simulink library "ConverterLibrary"  (R2026a)
settings: Solver=VariableStepAuto
undefined symbols (not defined in the file or in its folder): DiscIntNeverNeededParam, dspblkCoreblockFVToolHelper, gcbh, gridInverter
libraries: fl_lib x240, nesl_utility x221, ee_lib x208, slpidlib x28, eeGeneralControl x12, simulink x9, eeTransforms x4, simulink_extras x1, eePowerMeasurement x1
(part 10 of 30)

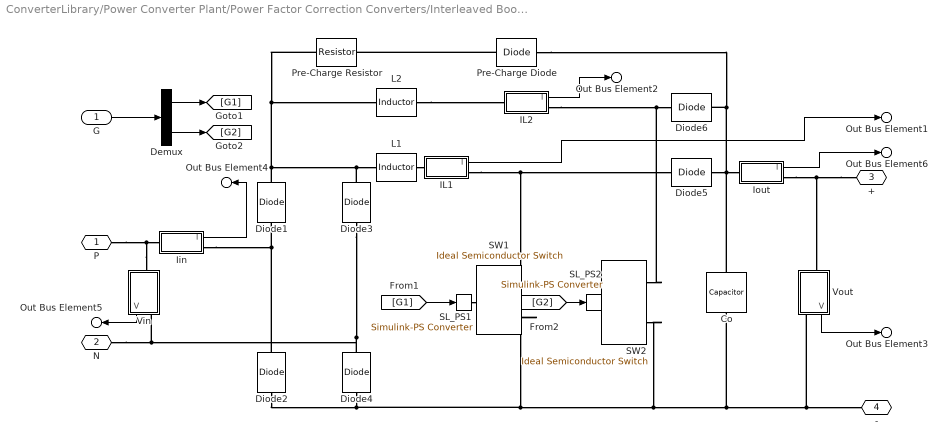
== system ConverterLibrary/Power Converter Plant/Power Factor Correction Converters/Interleaved Boost PFC Converter/InterleavedBoostPFCVariant/SimplifiedModel ==
  G : Inport
  Co : ee_lib/Passive/Capacitor  cap_option=ee.enum.passive.capacitor.capOption.const  c=CBoost_SI F  Cvec=[1e-05, 1e-06] F  Vvec=[0, 10] V  CV_table_symmetry=ee.enum.passive.capacitor.tableSymmetry.yes  f_vec=[1, 10] kHz  DFext_vec=[.8, 1.2]  enable_C_tol=ee.enum.toleranceApplication.none  averaging_period=0 s  C_tol=5  tol_distribution=ee.enum.toleranceDistribution.uniform  nSigma=4  r=Rco_SI Ohm  g=1e-05 1/Ohm  enable_operating_limits=ee.enum.enable.no  operating_limit_action=ee.enum.passive.reportOpLim.warn  max_working_voltage_range=[-25, 25] V  power_rating=1 W  maxTemperature=85 degC  thermalEnable=false  thermalMass=1 J/K  i_specify=off  i_priority=None  i=0 A  i_nominal_specify=off  i_nominal_value=1  i_nominal_unit=A  v_specify=off  v_priority=None  v=0 V  v_nominal_specify=off  v_nominal_value=1  v_nominal_unit=V  vc_specify=on  vc_priority=High  vc=Vco_SI V  vc_nominal_specify=off  vc_nominal_value=1  vc_nominal_unit=V  T_specify=off  T_priority=None  T=298.15 K  T_nominal_specify=off  T_nominal_value=1  T_nominal_unit=K
  Demux : Demux  Outputs=2
  Diode{1..4} (4 alike) : fl_lib/Electrical/Electrical Elements/Diode  Vf=VfRect_SI V  Ron=RdRect_SI Ohm  Goff=GdRect_SI 1/Ohm  i_specify=off  i_priority=None  i=0 A  i_nominal_specify=off  i_nominal_value=1  i_nominal_unit=A  v_specify=off  v_priority=None  v=0 V  v_nominal_specify=off  v_nominal_value=1  v_nominal_unit=V
  Diode5 : fl_lib/Electrical/Electrical Elements/Diode  Vf=VfDiode_SI V  Ron=RdDiode_SI Ohm  Goff=GdDiode_SI 1/Ohm  i_specify=off  i_priority=None  i=0 A  i_nominal_specify=off  i_nominal_value=1  i_nominal_unit=A  v_specify=off  v_priority=None  v=0 V  v_nominal_specify=off  v_nominal_value=1  v_nominal_unit=V
  Diode6 : fl_lib/Electrical/Electrical Elements/Diode  Vf=VfDiode_SI V  Ron=RdDiode_SI Ohm  Goff=GdDiode_SI 1/Ohm  i_specify=off  i_priority=None  i=0 A  i_nominal_specify=off  i_nominal_value=1  i_nominal_unit=A  v_specify=off  v_priority=None  v=0 V  v_nominal_specify=off  v_nominal_value=1  v_nominal_unit=V
  IL1 : Subsystem
      mask Display: disp('I')
  IL2 : Subsystem
      mask Display: disp('I')
  Iin : Subsystem
      mask Display: disp('I')
  Iout : Subsystem
      mask Display: disp('I')
  L1 : ee_lib/Passive/Inductor  l=LBoost_SI H  enable_L_tol=ee.enum.toleranceApplication.none  L_tol=20  tol_distribution=ee.enum.toleranceDistribution.uniform  nSigma=4  r=RLboost_SI Ohm  g=1e-05 1/Ohm  enable_operating_limits=ee.enum.enable.no  operating_limit_action=ee.enum.passive.reportOpLim.warn  max_working_current=1 A  power_rating=1 W  i_L_specify=off  i_L_priority=High  i_L=0 A  i_L_nominal_specify=off  i_L_nominal_value=1  i_L_nominal_unit=A
  L2 : ee_lib/Passive/Inductor  l=LBoost_SI H  enable_L_tol=ee.enum.toleranceApplication.none  L_tol=20  tol_distribution=ee.enum.toleranceDistribution.uniform  nSigma=4  r=RLboost_SI Ohm  g=1e-05 1/Ohm  enable_operating_limits=ee.enum.enable.no  operating_limit_action=ee.enum.passive.reportOpLim.warn  max_working_current=1 A  power_rating=1 W  i_L_specify=off  i_L_priority=High  i_L=0 A  i_L_nominal_specify=off  i_L_nominal_value=1  i_L_nominal_unit=A
  Pre-Charge Diode : fl_lib/Electrical/Electrical Elements/Diode  Vf=VfPreCharge_SI V  Ron=RdPreCharge_SI Ohm  Goff=GdPreCharge_SI 1/Ohm  i_specify=off  i_priority=None  i=0 A  i_nominal_specify=off  i_nominal_value=1  i_nominal_unit=A  v_specify=off  v_priority=None  v=0 V  v_nominal_specify=off  v_nominal_value=1  v_nominal_unit=V
  Pre-Charge Resistor : fl_lib/Electrical/Electrical Elements/Resistor  R=RPreCharge_SI Ohm  i_specify=off  i_priority=None  i=0 A  i_nominal_specify=off  i_nominal_value=1  i_nominal_unit=A  v_specify=off  v_priority=None  v=0 V  v_nominal_specify=off  v_nominal_value=1  v_nominal_unit=V
  SL_PS1 : nesl_utility/Simulink-PS Converter  PhysicalDomain=network_engine_domain  SubClassName=ps_input  LeftPortType=input  RightPortType=output  PseudoPeriodic=off  Frequencies=[]  NoiseDistribution=none  NoiseParameters=[]  Unit=1  AffineConversion=off  FilteringAndDerivatives=provide  SimscapeFilterOrder=1  InputFilterTimeConstant=0.001  UdotUserProvided=0
  SL_PS2 : nesl_utility/Simulink-PS Converter  PhysicalDomain=network_engine_domain  SubClassName=ps_input  LeftPortType=input  RightPortType=output  PseudoPeriodic=off  Frequencies=[]  NoiseDistribution=none  NoiseParameters=[]  Unit=1  AffineConversion=off  FilteringAndDerivatives=provide  SimscapeFilterOrder=1  InputFilterTimeConstant=0.001  UdotUserProvided=0
  SW1 : ee_lib/Semiconductors & Converters/Ideal Semiconductor Switch  port_option=ee.enum.controlport.ps  Ron=RdsOn_SI Ohm  Goff=GdsOff_SI 1/Ohm  Vth=Vth_SI V  diode_param=ee.enum.semiconductors.protectionDiode.external  diode_Vf=0.8 V  diode_Ron=0.001 Ohm  diode_Goff=1e-5 1/Ohm  diode_C=50e-9 F  diode_iRM=-235 A  diode_iF=300 A  diode_idot=-50 A/us  diode_trr_param=ee.enum.converters.diodetrr.trr_factor  diode_trr_factor=3  diode_trr=15 us  diode_Qrr=1500 s*uA
  SW2 : ee_lib/Semiconductors & Converters/Ideal Semiconductor Switch  port_option=ee.enum.controlport.ps  Ron=RdsOn_SI Ohm  Goff=GdsOff_SI 1/Ohm  Vth=Vth_SI V  diode_param=ee.enum.semiconductors.protectionDiode.external  diode_Vf=0.8 V  diode_Ron=0.001 Ohm  diode_Goff=1e-5 1/Ohm  diode_C=50e-9 F  diode_iRM=-235 A  diode_iF=300 A  diode_idot=-50 A/us  diode_trr_param=ee.enum.converters.diodetrr.trr_factor  diode_trr_factor=3  diode_trr=15 us  diode_Qrr=1500 s*uA
  Vin : Subsystem
      mask Display: disp('V')
  Vout : Subsystem
      settings: PortSchema="{\"entries\":[{\"content\":{\"sides\":[{\"content\":{\"connectorIds\":[\"LConn1\"]},\"type\":\"ConnectorPlacement.EquallySpacedRectSide\",\"uuid\":\"5f92137b-4b58-46b8-a68f-d3527484291c\"},{\"content\":{\"connectorIds\":[\"RConn1\",\"Out1\"],\"side\":\"RIGHT\"},\"type\":\"ConnectorPlacement.EquallySpacedRectSide\",\"uuid\":\"154b36f0-aa4a-4375-80c2-9c55af429c32\"},{\"content\":{\"side\":\"TOP\"},\"type\":\"ConnectorPlacement.EquallySpacedRectSide\",\"uuid\":\"6e01dd2b-817e-4c7e-a9bf-e017a248a3a8\"}]},\"type\":\"ConnectorPlacement.EquallySpacedConnector\",\"uuid\":\"a9d15cc4-68aa-466b-9599-7a273210f999\"}],\"packageUris\":[\"http://schema.mathworks.com/mf0/Connector/R2020b\"],\"version\":\"1.0\"}"
      mask Display: disp('V')
  P : PMIOPort  Side=Left
  N : PMIOPort  Port=2  Side=Left
  + : PMIOPort  Port=3  Side=Right
  - : PMIOPort  Port=4  Side=Right
  Out Bus Element1 : Outport  PortName=meas  Element=IL1 [A]
  Out Bus Element2 : Outport  PortName=meas  Element=IL2 [A]
  Out Bus Element3 : Outport  PortName=meas  Element=Vout [V]
  Out Bus Element4 : Outport  PortName=meas  Element=Iin [A]
  Out Bus Element5 : Outport  PortName=meas  Element=Vin [V]
  Out Bus Element6 : Outport  PortName=meas  Element=Iout [A]
  wires:
  [G2] -> SL_PS2/1
  IL2/1(I) -> Out Bus Element2/1
  IL1/1(I) -> Out Bus Element1/1
  Iout/1(I) -> Out Bus Element6/1
  Vin/1(V) -> Out Bus Element5/1
  Iin/1(I) -> Out Bus Element4/1
  Vout/1(V) -> Out Bus Element3/1
  [G1] -> SL_PS1/1
  Demux/2 -> [G2]
  Demux/1 -> [G1]
  G/1 -> Demux/1
  connections:
  SW2/LConn1 -- SL_PS2/RConn1
  Diode6/LConn1 -- SW2/RConn1 -- IL2/RConn1
  Vin/RConn1 -- N/RConn1 -- Diode3/LConn1 -- Diode4/RConn1
  Diode1/LConn1 -- Diode2/RConn1 -- Iin/RConn1
  +/RConn1 -- Vout/LConn1 -- Iout/RConn1
  Iout/LConn1 -- Co/LConn1 -- Pre-Charge Diode/RConn1 -- Diode6/RConn1 -- Diode5/RConn1
  L2/RConn1 -- IL2/LConn1
  SW1/RConn1 -- Diode5/LConn1 -- IL1/RConn1
  L1/RConn1 -- IL1/LConn1
  SW1/RConn2 -- SW2/RConn2 -- -/RConn1 -- Vout/RConn1 -- Co/RConn1 -- Diode2/LConn1 -- Diode4/LConn1
  Diode3/RConn1 -- L1/LConn1 -- Diode1/RConn1 -- Pre-Charge Resistor/LConn1 -- L2/LConn1
  Vin/LConn1 -- P/RConn1 -- Iin/LConn1
  SL_PS1/RConn1 -- SW1/LConn1
  Pre-Charge Diode/LConn1 -- Pre-Charge Resistor/RConn1

== system ConverterLibrary/Power Converter Plant/Power Factor Correction Converters/Totem-Pole Boost PFC Converter/TotemPoleBoostPFCVariant/DetailedModel ==
  G : Inport
  Co : ee_lib/Passive/Capacitor  cap_option=ee.enum.passive.capacitor.capOption.const  c=CBoost_SI F  Cvec=[1e-05, 1e-06] F  Vvec=[0, 10] V  CV_table_symmetry=ee.enum.passive.capacitor.tableSymmetry.yes  f_vec=[1, 10] kHz  DFext_vec=[.8, 1.2]  enable_C_tol=ee.enum.toleranceApplication.none  averaging_period=0 s  C_tol=5  tol_distribution=ee.enum.toleranceDistribution.uniform  nSigma=4  r=Rco_SI Ohm  g=1e-05 1/Ohm  enable_operating_limits=ee.enum.enable.no  operating_limit_action=ee.enum.passive.reportOpLim.warn  max_working_voltage_range=[-25, 25] V  power_rating=1 W  maxTemperature=85 degC  thermalEnable=false  thermalMass=1 J/K  i_specify=off  i_priority=None  i=0 A  i_nominal_specify=off  i_nominal_value=1  i_nominal_unit=A  v_specify=off  v_priority=None  v=0 V  v_nominal_specify=off  v_nominal_value=1  v_nominal_unit=V  vc_specify=on  vc_priority=High  vc=Vco_SI V  vc_nominal_specify=off  vc_nominal_value=1  vc_nominal_unit=V  T_specify=off  T_priority=None  T=298.15 K  T_nominal_specify=off  T_nominal_value=1  T_nominal_unit=K
  Demux : Demux
  FastLeg : Subsystem  Variant=on  VariantControlMode=label  LabelModeActiveChoice=SwitchingMOSFETwithThermal
      settings: PortSchema="{\"entries\":[{\"content\":{\"sides\":[{\"content\":{\"connectorIds\":[\"LConn1\",\"In1\"]},\"type\":\"ConnectorPlacement.EquallySpacedRectSide\",\"uuid\":\"77e2eceb-8f65-4ff8-b710-02732b9bb145\"},{\"content\":{\"connectorIds\":[\"RConn1\",\"RConn2\"],\"side\":\"RIGHT\"},\"type\":\"ConnectorPlacement.EquallySpacedRectSide\",\"uuid\":\"bfc7df5d-eb60-4c5b-86be-68c51cd3b8c3\"},{\"content\":{\"side\":\"TOP\"},\"type\":\"ConnectorPlacement.EquallySpacedRectSide\",\"uuid\":\"613efa33-60b7-4b5b-9311-a6c7287e5913\"}]},\"type\":\"ConnectorPlacement.EquallySpacedConnector\",\"uuid\":\"12746f96-860a-4c97-9f60-ace4c102aa63\"}],\"packageUris\":[\"http://schema.mathworks.com/mf0/Connector/R2020b\"],\"version\":\"1.0\"}"
  IL : Subsystem
      settings: PortSchema="{\"entries\":[{\"content\":{\"sides\":[{\"content\":{\"connectorIds\":[\"LConn1\"]},\"type\":\"ConnectorPlacement.EquallySpacedRectSide\",\"uuid\":\"80632e7e-66fe-49c8-894c-61cf7358e53a\"},{\"content\":{\"connectorIds\":[\"RConn1\"],\"side\":\"RIGHT\"},\"type\":\"ConnectorPlacement.EquallySpacedRectSide\",\"uuid\":\"7fb991d4-0257-47fa-8c16-238ff3f2e60c\"},{\"content\":{\"connectorIds\":[\"Out1\"],\"side\":\"TOP\"},\"type\":\"ConnectorPlacement.EquallySpacedRectSide\",\"uuid\":\"a2cf4f5e-7cb3-4577-a513-817a4fd9f07d\"}]},\"type\":\"ConnectorPlacement.EquallySpacedConnector\",\"uuid\":\"e3fac4ca-b917-4eeb-beb4-75837a4782c1\"}],\"packageUris\":[\"http://schema.mathworks.com/mf0/Connector/R2020b\"],\"version\":\"1.0\"}"
      mask Display: disp('I')
  Iout : Subsystem
      mask Display: disp('I')
  Lboost : ee_lib/Passive/Inductor  l=LBoost_SI H  enable_L_tol=ee.enum.toleranceApplication.none  L_tol=20  tol_distribution=ee.enum.toleranceDistribution.uniform  nSigma=4  r=RLboost_SI Ohm  g=1e-05 1/Ohm  enable_operating_limits=ee.enum.enable.no  operating_limit_action=ee.enum.passive.reportOpLim.warn  max_working_current=1 A  power_rating=1 W  i_L_specify=off  i_L_priority=High  i_L=0 A  i_L_nominal_specify=off  i_L_nominal_value=1  i_L_nominal_unit=A
  MuxFast : Mux  Inputs=2
  MuxSlow : Mux  Inputs=2
  SlowLeg : Subsystem  Variant=on  VariantControlMode=label  LabelModeActiveChoice=MOSFET
  Vin : Subsystem
      mask Display: disp('V')
  Vout : Subsystem
      settings: PortSchema="{\"entries\":[{\"content\":{\"sides\":[{\"content\":{\"connectorIds\":[\"LConn1\"]},\"type\":\"ConnectorPlacement.EquallySpacedRectSide\",\"uuid\":\"80632e7e-66fe-49c8-894c-61cf7358e53a\"},{\"content\":{\"connectorIds\":[\"RConn1\",\"Out1\"],\"side\":\"RIGHT\"},\"type\":\"ConnectorPlacement.EquallySpacedRectSide\",\"uuid\":\"7fb991d4-0257-47fa-8c16-238ff3f2e60c\"},{\"content\":{\"side\":\"TOP\"},\"type\":\"ConnectorPlacement.EquallySpacedRectSide\",\"uuid\":\"a2cf4f5e-7cb3-4577-a513-817a4fd9f07d\"}]},\"type\":\"ConnectorPlacement.EquallySpacedConnector\",\"uuid\":\"e3fac4ca-b917-4eeb-beb4-75837a4782c1\"}],\"packageUris\":[\"http://schema.mathworks.com/mf0/Connector/R2020b\"],\"version\":\"1.0\"}"
      mask Display: disp('V')
  P : PMIOPort  Side=Left
  N : PMIOPort  Port=2  Side=Left
  + : PMIOPort  Port=3  Side=Right
  - : PMIOPort  Port=4  Side=Right
  Out Bus Element1 : Outport  PortName=meas  Element=IL [A]
  Out Bus Element2 : Outport  PortName=meas  Element=Vout [V]
  Out Bus Element4 : Outport  PortName=meas  Element=Vin [V]
  Out Bus Element5 : Outport  PortName=meas  Element=Iout [A]
  wires:
  MuxFast/1 -> FastLeg/1(G)
  [G1] -> MuxFast/1
  [G2] -> MuxFast/2
  Vin/1(V) -> Out Bus Element4/1
  MuxSlow/1 -> SlowLeg/1(G)
  [G3] -> MuxSlow/1
  [G4] -> MuxSlow/2
  IL/1(I) -> Out Bus Element1/1
  Iout/1(I) -> Out Bus Element5/1  "Iout [A]"
  Vout/1(V) -> Out Bus Element2/1
  Demux/1 -> [G1]
  Demux/2 -> [G2]
  Demux/3 -> [G3]
  Demux/4 -> [G4]
  G/1 -> Demux/1
  connections:
  Lboost/LConn1 -- P/RConn1 -- Vin/LConn1
  SlowLeg/RConn1 -- FastLeg/RConn1 -- Co/LConn1 -- Iout/LConn1
  Lboost/RConn1 -- IL/LConn1
  Vin/RConn1 -- SlowLeg/LConn1 -- N/RConn1
  Iout/RConn1 -- Vout/LConn1 -- +/RConn1
  IL/RConn1 -- FastLeg/LConn1
  SlowLeg/RConn2 -- FastLeg/RConn2 -- Co/RConn1 -- -/RConn1 -- Vout/RConn1

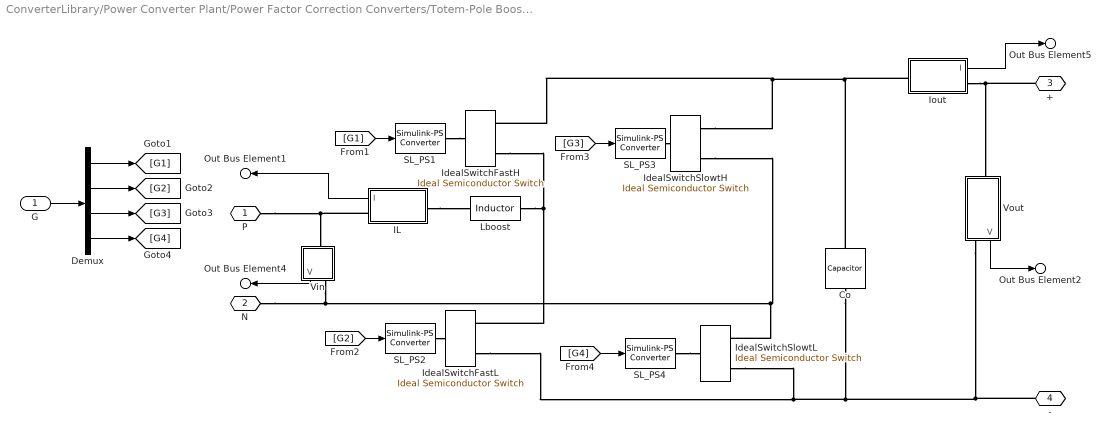
== system ConverterLibrary/Power Converter Plant/Power Factor Correction Converters/Totem-Pole Boost PFC Converter/TotemPoleBoostPFCVariant/SimplifiedModel ==
  G : Inport
  Co : ee_lib/Passive/Capacitor  cap_option=ee.enum.passive.capacitor.capOption.const  c=CBoost_SI F  Cvec=[1e-05, 1e-06] F  Vvec=[0, 10] V  CV_table_symmetry=ee.enum.passive.capacitor.tableSymmetry.yes  f_vec=[1, 10] kHz  DFext_vec=[.8, 1.2]  enable_C_tol=ee.enum.toleranceApplication.none  averaging_period=0 s  C_tol=5  tol_distribution=ee.enum.toleranceDistribution.uniform  nSigma=4  r=Rco_SI Ohm  g=1e-05 1/Ohm  enable_operating_limits=ee.enum.enable.no  operating_limit_action=ee.enum.passive.reportOpLim.warn  max_working_voltage_range=[-25, 25] V  power_rating=1 W  maxTemperature=85 degC  thermalEnable=false  thermalMass=1 J/K  i_specify=off  i_priority=None  i=0 A  i_nominal_specify=off  i_nominal_value=1  i_nominal_unit=A  v_specify=off  v_priority=None  v=0 V  v_nominal_specify=off  v_nominal_value=1  v_nominal_unit=V  vc_specify=on  vc_priority=High  vc=Vco_SI V  vc_nominal_specify=off  vc_nominal_value=1  vc_nominal_unit=V  T_specify=off  T_priority=None  T=298.15 K  T_nominal_specify=off  T_nominal_value=1  T_nominal_unit=K
  Demux : Demux
  IL : Subsystem
      settings: PortSchema="{\"entries\":[{\"content\":{\"sides\":[{\"content\":{\"connectorIds\":[\"Out1\",\"LConn1\"]},\"type\":\"ConnectorPlacement.EquallySpacedRectSide\",\"uuid\":\"39b7e526-9a68-4c73-9ad6-fd149fea363a\"},{\"content\":{\"connectorIds\":[\"RConn1\"],\"side\":\"RIGHT\"},\"type\":\"ConnectorPlacement.EquallySpacedRectSide\",\"uuid\":\"ee3f62d2-02c4-4290-ad83-c24a9e891d89\"},{\"content\":{\"side\":\"TOP\"},\"type\":\"ConnectorPlacement.EquallySpacedRectSide\",\"uuid\":\"a8618696-d9d3-41f8-b97f-996b903ae337\"}]},\"type\":\"ConnectorPlacement.EquallySpacedConnector\",\"uuid\":\"57ec1f0b-c67f-47bc-9e24-5102208e6cfb\"}],\"packageUris\":[\"http://schema.mathworks.com/mf0/Connector/R2020b\"],\"version\":\"1.0\"}"
      mask Display: disp('I')
  IdealSwitchFastH : ee_lib/Semiconductors & Converters/Ideal Semiconductor Switch  port_option=ee.enum.controlport.ps  Ron=RdsOnFast_SI Ohm  Goff=GdsOffFast_SI 1/Ohm  Vth=VthFast_SI V  diode_param=ee.enum.semiconductors.protectionDiode.nodynamics  diode_Vf=VfFast_SI V  diode_Ron=RdFast_SI Ohm  diode_Goff=GdFast_SI 1/Ohm  diode_C=50e-9 F  diode_iRM=-235 A  diode_iF=300 A  diode_idot=-50 A/us  diode_trr_param=ee.enum.converters.diodetrr.trr_factor  diode_trr_factor=3  diode_trr=15 us  diode_Qrr=1500 s*uA
  IdealSwitchFastL : ee_lib/Semiconductors & Converters/Ideal Semiconductor Switch  port_option=ee.enum.controlport.ps  Ron=RdsOnFast_SI Ohm  Goff=GdsOffFast_SI 1/Ohm  Vth=VthFast_SI V  diode_param=ee.enum.semiconductors.protectionDiode.nodynamics  diode_Vf=VfFast_SI V  diode_Ron=RdFast_SI Ohm  diode_Goff=GdFast_SI 1/Ohm  diode_C=50e-9 F  diode_iRM=-235 A  diode_iF=300 A  diode_idot=-50 A/us  diode_trr_param=ee.enum.converters.diodetrr.trr_factor  diode_trr_factor=3  diode_trr=15 us  diode_Qrr=1500 s*uA
  IdealSwitchSlowtH : ee_lib/Semiconductors & Converters/Ideal Semiconductor Switch  port_option=ee.enum.controlport.ps  Ron=RdsOnSlow_SI Ohm  Goff=GdsOffSlow_SI 1/Ohm  Vth=VthSlow_SI V  diode_param=ee.enum.semiconductors.protectionDiode.nodynamics  diode_Vf=VfSlow_SI V  diode_Ron=RdSlow_SI Ohm  diode_Goff=GdSlow_SI 1/Ohm  diode_C=50e-9 F  diode_iRM=-235 A  diode_iF=300 A  diode_idot=-50 A/us  diode_trr_param=ee.enum.converters.diodetrr.trr_factor  diode_trr_factor=3  diode_trr=15 us  diode_Qrr=1500 s*uA
  IdealSwitchSlowtL : ee_lib/Semiconductors & Converters/Ideal Semiconductor Switch  port_option=ee.enum.controlport.ps  Ron=RdsOnSlow_SI Ohm  Goff=GdsOffSlow_SI 1/Ohm  Vth=VthSlow_SI V  diode_param=ee.enum.semiconductors.protectionDiode.nodynamics  diode_Vf=VfSlow_SI V  diode_Ron=RdSlow_SI Ohm  diode_Goff=GdSlow_SI 1/Ohm  diode_C=50e-9 F  diode_iRM=-235 A  diode_iF=300 A  diode_idot=-50 A/us  diode_trr_param=ee.enum.converters.diodetrr.trr_factor  diode_trr_factor=3  diode_trr=15 us  diode_Qrr=1500 s*uA
  Iout : Subsystem
      mask Display: disp('I')
  Lboost : ee_lib/Passive/Inductor  l=LBoost_SI H  enable_L_tol=ee.enum.toleranceApplication.none  L_tol=20  tol_distribution=ee.enum.toleranceDistribution.uniform  nSigma=4  r=RLboost_SI Ohm  g=1e-05 1/Ohm  enable_operating_limits=ee.enum.enable.no  operating_limit_action=ee.enum.passive.reportOpLim.warn  max_working_current=1 A  power_rating=1 W  i_L_specify=off  i_L_priority=High  i_L=0 A  i_L_nominal_specify=off  i_L_nominal_value=1  i_L_nominal_unit=A
  SL_PS{1..4} (4 alike) : nesl_utility/Simulink-PS Converter  PhysicalDomain=network_engine_domain  SubClassName=ps_input  LeftPortType=input  RightPortType=output  PseudoPeriodic=off  Frequencies=[]  NoiseDistribution=none  NoiseParameters=[]  Unit=1  AffineConversion=off  FilteringAndDerivatives=provide  SimscapeFilterOrder=1  InputFilterTimeConstant=0.001  UdotUserProvided=0
  Vin : Subsystem
      mask Display: disp('V')
  Vout : Subsystem
      settings: PortSchema="{\"entries\":[{\"content\":{\"sides\":[{\"content\":{\"connectorIds\":[\"LConn1\"]},\"type\":\"ConnectorPlacement.EquallySpacedRectSide\",\"uuid\":\"39b7e526-9a68-4c73-9ad6-fd149fea363a\"},{\"content\":{\"connectorIds\":[\"RConn1\",\"Out1\"],\"side\":\"RIGHT\"},\"type\":\"ConnectorPlacement.EquallySpacedRectSide\",\"uuid\":\"ee3f62d2-02c4-4290-ad83-c24a9e891d89\"},{\"content\":{\"side\":\"TOP\"},\"type\":\"ConnectorPlacement.EquallySpacedRectSide\",\"uuid\":\"a8618696-d9d3-41f8-b97f-996b903ae337\"}]},\"type\":\"ConnectorPlacement.EquallySpacedConnector\",\"uuid\":\"57ec1f0b-c67f-47bc-9e24-5102208e6cfb\"}],\"packageUris\":[\"http://schema.mathworks.com/mf0/Connector/R2020b\"],\"version\":\"1.0\"}"
      mask Display: disp('V')
  P : PMIOPort  Side=Left
  N : PMIOPort  Port=2  Side=Left
  + : PMIOPort  Port=3  Side=Right
  - : PMIOPort  Port=4  Side=Right
  Out Bus Element1 : Outport  PortName=meas  Element=IL [A]
  Out Bus Element2 : Outport  PortName=meas  Element=Vout [V]
  Out Bus Element4 : Outport  PortName=meas  Element=Vin [V]
  Out Bus Element5 : Outport  PortName=meas  Element=Iout [A]
  wires:
  G/1 -> Demux/1
  Demux/1 -> [G1]
  Demux/2 -> [G2]
  Demux/3 -> [G3]
  Demux/4 -> [G4]
  [G1] -> SL_PS1/1
  [G2] -> SL_PS2/1
  [G3] -> SL_PS3/1
  [G4] -> SL_PS4/1
  IL/1(I) -> Out Bus Element1/1
  Vout/1(V) -> Out Bus Element2/1
  Vin/1(V) -> Out Bus Element4/1
  Iout/1(I) -> Out Bus Element5/1
  connections:
  Lboost/RConn1 -- IdealSwitchFastL/RConn1 -- IdealSwitchFastH/RConn2
  SL_PS1/RConn1 -- IdealSwitchFastH/LConn1
  SL_PS2/RConn1 -- IdealSwitchFastL/LConn1
  IL/LConn1 -- P/RConn1 -- Vin/LConn1
  IdealSwitchFastL/RConn2 -- IdealSwitchSlowtL/RConn2 -- Co/RConn1 -- Vout/RConn1 -- -/RConn1
  Iout/RConn1 -- Vout/LConn1 -- +/RConn1
  IL/RConn1 -- Lboost/LConn1
  IdealSwitchFastH/RConn1 -- IdealSwitchSlowtH/RConn1 -- Iout/LConn1 -- Co/LConn1
  SL_PS3/RConn1 -- IdealSwitchSlowtH/LConn1
  SL_PS4/RConn1 -- IdealSwitchSlowtL/LConn1
  IdealSwitchSlowtL/RConn1 -- IdealSwitchSlowtH/RConn2 -- N/RConn1 -- Vin/RConn1

== system ConverterLibrary/Power Converter Plant/Soft-Switching Converters/CLLC Converter/CLLCConverterVariant/DetailedModel ==
  Gpri : Inport
  Gsec : Inport  Port=2
  Bus Creator : BusCreator  Inputs=3
  Primary Converter : Subsystem
      settings: PortSchema="{\"entries\":[{\"content\":{\"sides\":[{\"content\":{\"connectorIds\":[\"LConn1\",\"LConn2\"]},\"type\":\"ConnectorPlacement.EquallySpacedRectSide\",\"uuid\":\"5f98eff0-54e4-47a8-aeeb-0279cba14f26\"},{\"content\":{\"connectorIds\":[\"RConn1\",\"RConn2\"],\"side\":\"RIGHT\"},\"type\":\"ConnectorPlacement.EquallySpacedRectSide\",\"uuid\":\"71acbbb6-1fc8-426c-b389-5d494eb18bfd\"},{\"content\":{\"connectorIds\":[\"In1\",\"Out1\"],\"side\":\"TOP\"},\"type\":\"ConnectorPlacement.EquallySpacedRectSide\",\"uuid\":\"dc77ee05-1f57-4323-bfda-b0076e2d1ee5\"}]},\"type\":\"ConnectorPlacement.EquallySpacedConnector\",\"uuid\":\"8d0b8c05-d5c5-4033-af60-ebdb639bdc40\"}],\"packageUris\":[\"http://schema.mathworks.com/mf0/Connector/R2020b\"],\"version\":\"1.0\"}"
  Resonant Tank : Subsystem
      settings: PortSchema="{\"entries\":[{\"content\":{\"sides\":[{\"content\":{\"connectorIds\":[\"LConn1\",\"LConn2\"]},\"type\":\"ConnectorPlacement.EquallySpacedRectSide\",\"uuid\":\"d505f362-3b8e-4dee-9b5b-731d75550efb\"},{\"content\":{\"connectorIds\":[\"RConn1\",\"RConn2\"],\"side\":\"RIGHT\"},\"type\":\"ConnectorPlacement.EquallySpacedRectSide\",\"uuid\":\"66ab4b84-9b7a-404b-b3f6-3ac1c371ea42\"},{\"content\":{\"connectorIds\":[\"Out1\"],\"side\":\"TOP\"},\"type\":\"ConnectorPlacement.EquallySpacedRectSide\",\"uuid\":\"00605859-d490-4a3b-aace-391362dfba7e\"}]},\"type\":\"ConnectorPlacement.EquallySpacedConnector\",\"uuid\":\"a210fe68-7181-499f-8e1c-ccfe71b42a4c\"}],\"packageUris\":[\"http://schema.mathworks.com/mf0/Connector/R2020b\"],\"version\":\"1.0\"}"
      mask Display: image('CLLCTransformerIcon.png');
  Secondary Converter : Subsystem
      settings: PortSchema="{\"entries\":[{\"content\":{\"sides\":[{\"content\":{\"connectorIds\":[\"LConn1\",\"LConn2\"]},\"type\":\"ConnectorPlacement.EquallySpacedRectSide\",\"uuid\":\"4786b3cc-2245-4c72-a50b-9c63e4ad3d8a\"},{\"content\":{\"connectorIds\":[\"RConn1\",\"RConn2\"],\"side\":\"RIGHT\"},\"type\":\"ConnectorPlacement.EquallySpacedRectSide\",\"uuid\":\"250a01d0-bf95-4e01-bf69-d866bcf3b7bd\"},{\"content\":{\"connectorIds\":[\"In1\",\"Out1\"],\"side\":\"TOP\"},\"type\":\"ConnectorPlacement.EquallySpacedRectSide\",\"uuid\":\"52730d18-084b-4644-8b2a-b54c84fa88ec\"}]},\"type\":\"ConnectorPlacement.EquallySpacedConnector\",\"uuid\":\"d24cae2a-f132-4f5a-ac35-d7440d7a99e9\"}],\"packageUris\":[\"http://schema.mathworks.com/mf0/Connector/R2020b\"],\"version\":\"1.0\"}"
  P1 : PMIOPort  Side=Left
  P2 : PMIOPort  Port=2  Side=Right
  N1 : PMIOPort  Port=3  Side=Left
  N2 : PMIOPort  Port=4  Side=Right
  Meas : Outport
  wires:
  Resonant Tank/1(meas) -> Bus Creator/2  "ResonantTank"
  Bus Creator/1 -> Meas/1
  Secondary Converter/1(meas) -> Bus Creator/3  "Rectifier"
  Primary Converter/1(meas) -> Bus Creator/1  "Inverter"
  Gsec/1 -> Secondary Converter/1(G)
  Gpri/1 -> Primary Converter/1(G)
  connections:
  Resonant Tank/RConn1 -- Secondary Converter/LConn1
  Resonant Tank/LConn2 -- Primary Converter/RConn2
  P2/RConn1 -- Secondary Converter/RConn1
  P1/RConn1 -- Primary Converter/LConn1
  Resonant Tank/RConn2 -- Secondary Converter/LConn2
  Resonant Tank/LConn1 -- Primary Converter/RConn1
  N2/RConn1 -- Secondary Converter/RConn2
  N1/RConn1 -- Primary Converter/LConn2

== system ConverterLibrary/Power Converter Plant/Soft-Switching Converters/CLLC Converter/CLLCConverterVariant/SimplifiedModel ==
  Gpri : Inport
  Gsec : Inport  Port=2
  Bus Creator : BusCreator  Inputs=3
  Primary Converter : Subsystem
      settings: PortSchema="{\"entries\":[{\"content\":{\"sides\":[{\"content\":{\"connectorIds\":[\"LConn1\",\"LConn2\"]},\"type\":\"ConnectorPlacement.EquallySpacedRectSide\",\"uuid\":\"5f98eff0-54e4-47a8-aeeb-0279cba14f26\"},{\"content\":{\"connectorIds\":[\"RConn1\",\"RConn2\"],\"side\":\"RIGHT\"},\"type\":\"ConnectorPlacement.EquallySpacedRectSide\",\"uuid\":\"71acbbb6-1fc8-426c-b389-5d494eb18bfd\"},{\"content\":{\"connectorIds\":[\"In1\",\"Out1\"],\"side\":\"TOP\"},\"type\":\"ConnectorPlacement.EquallySpacedRectSide\",\"uuid\":\"dc77ee05-1f57-4323-bfda-b0076e2d1ee5\"}]},\"type\":\"ConnectorPlacement.EquallySpacedConnector\",\"uuid\":\"8d0b8c05-d5c5-4033-af60-ebdb639bdc40\"}],\"packageUris\":[\"http://schema.mathworks.com/mf0/Connector/R2020b\"],\"version\":\"1.0\"}"
  Resonant Tank : Subsystem
      settings: PortSchema="{\"entries\":[{\"content\":{\"sides\":[{\"content\":{\"connectorIds\":[\"LConn1\",\"LConn2\"]},\"type\":\"ConnectorPlacement.EquallySpacedRectSide\",\"uuid\":\"d505f362-3b8e-4dee-9b5b-731d75550efb\"},{\"content\":{\"connectorIds\":[\"RConn1\",\"RConn2\"],\"side\":\"RIGHT\"},\"type\":\"ConnectorPlacement.EquallySpacedRectSide\",\"uuid\":\"66ab4b84-9b7a-404b-b3f6-3ac1c371ea42\"},{\"content\":{\"connectorIds\":[\"Out1\"],\"side\":\"TOP\"},\"type\":\"ConnectorPlacement.EquallySpacedRectSide\",\"uuid\":\"00605859-d490-4a3b-aace-391362dfba7e\"}]},\"type\":\"ConnectorPlacement.EquallySpacedConnector\",\"uuid\":\"a210fe68-7181-499f-8e1c-ccfe71b42a4c\"}],\"packageUris\":[\"http://schema.mathworks.com/mf0/Connector/R2020b\"],\"version\":\"1.0\"}"
      mask Display: image('CLLCTransformerIcon.png');
  Secondary Converter : Subsystem
      settings: PortSchema="{\"entries\":[{\"content\":{\"sides\":[{\"content\":{\"connectorIds\":[\"LConn1\",\"LConn2\"]},\"type\":\"ConnectorPlacement.EquallySpacedRectSide\",\"uuid\":\"4786b3cc-2245-4c72-a50b-9c63e4ad3d8a\"},{\"content\":{\"connectorIds\":[\"RConn1\",\"RConn2\"],\"side\":\"RIGHT\"},\"type\":\"ConnectorPlacement.EquallySpacedRectSide\",\"uuid\":\"250a01d0-bf95-4e01-bf69-d866bcf3b7bd\"},{\"content\":{\"connectorIds\":[\"In1\",\"Out1\"],\"side\":\"TOP\"},\"type\":\"ConnectorPlacement.EquallySpacedRectSide\",\"uuid\":\"52730d18-084b-4644-8b2a-b54c84fa88ec\"}]},\"type\":\"ConnectorPlacement.EquallySpacedConnector\",\"uuid\":\"d24cae2a-f132-4f5a-ac35-d7440d7a99e9\"}],\"packageUris\":[\"http://schema.mathworks.com/mf0/Connector/R2020b\"],\"version\":\"1.0\"}"
  P1 : PMIOPort  Side=Left
  P2 : PMIOPort  Port=2  Side=Right
  N1 : PMIOPort  Port=3  Side=Left
  N2 : PMIOPort  Port=4  Side=Right
  Meas : Outport
  wires:
  Gpri/1 -> Primary Converter/1(G)
  Gsec/1 -> Secondary Converter/1(G)
  Primary Converter/1(meas) -> Bus Creator/1  "Inverter"
  Secondary Converter/1(meas) -> Bus Creator/3  "Rectifier"
  Bus Creator/1 -> Meas/1
  Resonant Tank/1(meas) -> Bus Creator/2  "ResonantTank"
  connections:
  N1/RConn1 -- Primary Converter/LConn2
  N2/RConn1 -- Secondary Converter/RConn2
  Resonant Tank/LConn1 -- Primary Converter/RConn1
  Resonant Tank/RConn2 -- Secondary Converter/LConn2
  P1/RConn1 -- Primary Converter/LConn1
  P2/RConn1 -- Secondary Converter/RConn1
  Resonant Tank/LConn2 -- Primary Converter/RConn2
  Resonant Tank/RConn1 -- Secondary Converter/LConn1

== system ConverterLibrary/Power Converter Plant/Soft-Switching Converters/DAB Converter/DABConverterVariant/DetailedModel ==
  Gp : Inport
  Gs : Inport  Port=2
  Co : ee_lib/Passive/Capacitor  cap_option=ee.enum.passive.capacitor.capOption.const  c=Co_SI F  Cvec=[1e-05, 1e-06] F  Vvec=[0, 10] V  CV_table_symmetry=ee.enum.passive.capacitor.tableSymmetry.yes  f_vec=[1, 10] kHz  DFext_vec=[.8, 1.2]  enable_C_tol=ee.enum.toleranceApplication.none  averaging_period=0 s  C_tol=5  tol_distribution=ee.enum.toleranceDistribution.uniform  nSigma=4  r=Rco_SI Ohm  g=1e-05 1/Ohm  enable_operating_limits=ee.enum.enable.no  operating_limit_action=ee.enum.passive.reportOpLim.warn  max_working_voltage_range=[-25, 25] V  power_rating=1 W  maxTemperature=85 degC  thermalEnable=false  thermalMass=1 J/K  i_specify=off  i_priority=None  i=0 A  i_nominal_specify=off  i_nominal_value=1  i_nominal_unit=A  v_specify=off  v_priority=None  v=0 V  v_nominal_specify=off  v_nominal_value=1  v_nominal_unit=V  vc_specify=on  vc_priority=High  vc=Vco_SI V  vc_nominal_specify=off  vc_nominal_value=1  vc_nominal_unit=V  T_specify=off  T_priority=None  T=298.15 K  T_nominal_specify=off  T_nominal_value=1  T_nominal_unit=K
  Iin : Subsystem
      mask Display: disp('I')
  Iout : Subsystem
      mask Display: disp('I')
  Ip : Subsystem
      mask Display: disp('I')
  Is : Subsystem
      settings: PortSchema="{\"entries\":[{\"content\":{\"sides\":[{\"content\":{\"connectorIds\":[\"Out1\",\"LConn1\"]},\"type\":\"ConnectorPlacement.EquallySpacedRectSide\",\"uuid\":\"da66b42d-39ba-4e5d-9b19-dc680792542d\"},{\"content\":{\"connectorIds\":[\"RConn1\"],\"side\":\"RIGHT\"},\"type\":\"ConnectorPlacement.EquallySpacedRectSide\",\"uuid\":\"9a34d54a-b1f0-405a-82c9-4333c7864e33\"},{\"content\":{\"side\":\"TOP\"},\"type\":\"ConnectorPlacement.EquallySpacedRectSide\",\"uuid\":\"3d98f795-d173-4072-aa84-47617691d0d7\"}]},\"type\":\"ConnectorPlacement.EquallySpacedConnector\",\"uuid\":\"cc1a3107-18f6-4c4b-a82f-56637250e4a4\"}],\"packageUris\":[\"http://schema.mathworks.com/mf0/Connector/R2020b\"],\"version\":\"1.0\"}"
      mask Display: disp('I')
  Lr : Subsystem  Variant=on  VariantControlMode=label  LabelModeActiveChoice=LeakageInductance
  Nonlinear Transformer : ee_lib/Passive/Transformers/Nonlinear Transformer  Nw=turnsRatio  Nw2=1  winding_param_option=2  Req=0.001 Ohm  Leq=0 H  R_1=RLlk1_SI Ohm  L_1=Llk1_SI H  R_2=RLlk2_SI Ohm  L_2=Llk2_SI H  averaging_period=0 s  R_m=15000 Ohm  parameterization_option=1  H_data=[0, 200, 400, 600, 800, 1000] A/m  B_data=[0, .81, 1.25, 1.42, 1.48, 1.49] T  length_effective=0.2 m  area_effective=2e-4 m^2  L=Lm_SI H  L_sat=1e-2 H  current_data=[0, .4, .8, 1.2, 1.6, 2] A  magnetic_flux_data=[0, .161, .25, .284, .295, .299] .* 1e-3 Wb  magnetic_flux_sat=1.6e-04 Wb  dBdH0=0.005 T*m/A  B1=1.49 T  H1=1000 A/m  c=0.1  K=200 A/m  alpha=1e-4  interpolation_option=1  Leq_i0=0 A  L1_i0=0 A  L2_i0=0 A  x0_option=1  i_L0=0 A  phi0=0 Wb  B0=0 T  H0=0 A/m  Leq_g=1e-05 1/Ohm  L1_g=1e-05 1/Ohm  L2_g=1e-05 1/Ohm
  PrimaryBridge : Subsystem  Variant=on  VariantControlMode=label  LabelModeActiveChoice=SwitchingMOSFETwithThermal
      settings: PortSchema="{\"entries\":[{\"content\":{\"sides\":[{\"content\":{\"connectorIds\":[\"LConn1\",\"LConn2\"]},\"type\":\"ConnectorPlacement.EquallySpacedRectSide\",\"uuid\":\"d98ab02e-eaff-433c-abe3-9c8832e30ad4\"},{\"content\":{\"connectorIds\":[\"RConn1\",\"RConn2\"],\"side\":\"RIGHT\"},\"type\":\"ConnectorPlacement.EquallySpacedRectSide\",\"uuid\":\"c0772040-dd18-4215-ab8f-2785b86fdc85\"},{\"content\":{\"connectorIds\":[\"In1\"],\"side\":\"TOP\"},\"type\":\"ConnectorPlacement.EquallySpacedRectSide\",\"uuid\":\"58c66fea-5b87-40d4-9fd7-49b3eaec4a75\"}]},\"type\":\"ConnectorPlacement.EquallySpacedConnector\",\"uuid\":\"277158f2-ac55-4232-8e6b-6b9d1c92778d\"}],\"packageUris\":[\"http://schema.mathworks.com/mf0/Connector/R2020b\"],\"version\":\"1.0\"}"
  SecondaryBridge : Subsystem  Variant=on  VariantControlMode=label  LabelModeActiveChoice=SwitchingMOSFETwithThermal
      settings: PortSchema="{\"entries\":[{\"content\":{\"sides\":[{\"content\":{\"connectorIds\":[\"LConn1\",\"LConn2\"]},\"type\":\"ConnectorPlacement.EquallySpacedRectSide\",\"uuid\":\"d98ab02e-eaff-433c-abe3-9c8832e30ad4\"},{\"content\":{\"connectorIds\":[\"RConn1\",\"RConn2\"],\"side\":\"RIGHT\"},\"type\":\"ConnectorPlacement.EquallySpacedRectSide\",\"uuid\":\"c0772040-dd18-4215-ab8f-2785b86fdc85\"},{\"content\":{\"connectorIds\":[\"In1\"],\"side\":\"TOP\"},\"type\":\"ConnectorPlacement.EquallySpacedRectSide\",\"uuid\":\"58c66fea-5b87-40d4-9fd7-49b3eaec4a75\"}]},\"type\":\"ConnectorPlacement.EquallySpacedConnector\",\"uuid\":\"277158f2-ac55-4232-8e6b-6b9d1c92778d\"}],\"packageUris\":[\"http://schema.mathworks.com/mf0/Connector/R2020b\"],\"version\":\"1.0\"}"
  Vin : Subsystem
      mask Display: disp('V')
  Vout : Subsystem
      settings: PortSchema="{\"entries\":[{\"content\":{\"sides\":[{\"content\":{\"connectorIds\":[\"LConn1\"]},\"type\":\"ConnectorPlacement.EquallySpacedRectSide\",\"uuid\":\"da66b42d-39ba-4e5d-9b19-dc680792542d\"},{\"content\":{\"connectorIds\":[\"RConn1\",\"Out1\"],\"side\":\"RIGHT\"},\"type\":\"ConnectorPlacement.EquallySpacedRectSide\",\"uuid\":\"9a34d54a-b1f0-405a-82c9-4333c7864e33\"},{\"content\":{\"side\":\"TOP\"},\"type\":\"ConnectorPlacement.EquallySpacedRectSide\",\"uuid\":\"3d98f795-d173-4072-aa84-47617691d0d7\"}]},\"type\":\"ConnectorPlacement.EquallySpacedConnector\",\"uuid\":\"cc1a3107-18f6-4c4b-a82f-56637250e4a4\"}],\"packageUris\":[\"http://schema.mathworks.com/mf0/Connector/R2020b\"],\"version\":\"1.0\"}"
      mask Display: disp('V')
  Vin+ : PMIOPort  Side=Left
  Vin- : PMIOPort  Port=2  Side=Left
  Vout+ : PMIOPort  Port=3  Side=Right
  Vout- : PMIOPort  Port=4  Side=Right
  Out Bus Element1 : Outport  PortName=meas  Element=Ip [A]
  Out Bus Element2 : Outport  PortName=meas  Element=Is [A]
  Out Bus Element3 : Outport  PortName=meas  Element=Vin [V]
  Out Bus Element4 : Outport  PortName=meas  Element=Vout [V]
  Out Bus Element5 : Outport  PortName=meas  Element=Iin [A]
  Out Bus Element6 : Outport  PortName=meas  Element=Iout [A]
  wires:
  Gp/1 -> PrimaryBridge/1(G)
  Gs/1 -> SecondaryBridge/1(G)
  Vout/1(V) -> Out Bus Element4/1  "Vout [V]"
  Is/1(I) -> Out Bus Element2/1
  Iout/1(I) -> Out Bus Element6/1
  Iin/1(I) -> Out Bus Element5/1  "Iin [A]"
  Vin/1(V) -> Out Bus Element3/1  "Vin [V]"
  Ip/1(I) -> Out Bus Element1/1  "Ip [A]"
  connections:
  Co/LConn1 -- SecondaryBridge/LConn1 -- Iout/LConn1
  Vout-/RConn1 -- SecondaryBridge/LConn2 -- Co/RConn1 -- Vout/RConn1
  Iin/LConn1 -- Vin+/RConn1 -- Vin/LConn1
  Vin/RConn1 -- Vin-/RConn1 -- PrimaryBridge/LConn2
  Vout+/RConn1 -- Vout/LConn1 -- Iout/RConn1
  Nonlinear Transformer/RConn1 -- Is/LConn1
  Nonlinear Transformer/LConn2 -- PrimaryBridge/RConn2
  Nonlinear Transformer/LConn1 -- Lr/RConn1
  Lr/LConn1 -- Ip/RConn1
  PrimaryBridge/RConn1 -- Ip/LConn1
  Iin/RConn1 -- PrimaryBridge/LConn1
  Is/RConn1 -- SecondaryBridge/RConn1
  Nonlinear Transformer/RConn2 -- SecondaryBridge/RConn2

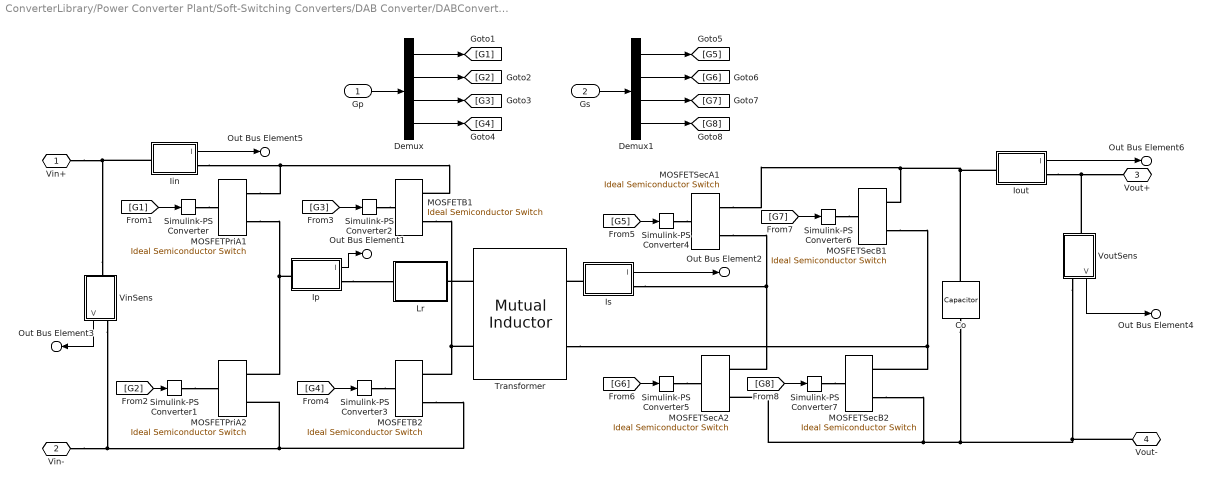
== system ConverterLibrary/Power Converter Plant/Soft-Switching Converters/DAB Converter/DABConverterVariant/SimplifiedModel ==
  Gp : Inport
  Gs : Inport  Port=2
  Co : ee_lib/Passive/Capacitor  cap_option=ee.enum.passive.capacitor.capOption.const  c=Co_SI F  Cvec=[1e-05, 1e-06] F  Vvec=[0, 10] V  CV_table_symmetry=ee.enum.passive.capacitor.tableSymmetry.yes  f_vec=[1, 10] kHz  DFext_vec=[.8, 1.2]  enable_C_tol=ee.enum.toleranceApplication.none  averaging_period=0 s  C_tol=5  tol_distribution=ee.enum.toleranceDistribution.uniform  nSigma=4  r=Rco_SI Ohm  g=1e-05 1/Ohm  enable_operating_limits=ee.enum.enable.no  operating_limit_action=ee.enum.passive.reportOpLim.warn  max_working_voltage_range=[-25, 25] V  power_rating=1 W  maxTemperature=85 degC  thermalEnable=false  thermalMass=1 J/K  i_specify=off  i_priority=None  i=0 A  i_nominal_specify=off  i_nominal_value=1  i_nominal_unit=A  v_specify=off  v_priority=None  v=0 V  v_nominal_specify=off  v_nominal_value=1  v_nominal_unit=V  vc_specify=on  vc_priority=High  vc=Vco_SI V  vc_nominal_specify=off  vc_nominal_value=1  vc_nominal_unit=V  T_specify=off  T_priority=None  T=298.15 K  T_nominal_specify=off  T_nominal_value=1  T_nominal_unit=K
  Demux : Demux
  Demux1 : Demux
  Iin : Subsystem
      mask Display: disp('I')
  Iout : Subsystem
      mask Display: disp('I')
  Ip : Subsystem
      mask Display: disp('I')
  Is : Subsystem
      mask Display: disp('I')
  Lr : Subsystem  Variant=on  VariantControlMode=label  LabelModeActiveChoice=LeakageInductance
  MOSFETB1 : ee_lib/Semiconductors & Converters/Ideal Semiconductor Switch  port_option=ee.enum.controlport.ps  Ron=RdsOnPri_SI Ohm  Goff=GdsOffPri_SI 1/Ohm  Vth=VthPri_SI V  diode_param=ee.enum.semiconductors.protectionDiode.nodynamics  diode_Vf=VfPri_SI V  diode_Ron=RdPri_SI Ohm  diode_Goff=GdPri_SI 1/Ohm  diode_C=50e-9 F  diode_iRM=-235 A  diode_iF=300 A  diode_idot=-50 A/us  diode_trr_param=ee.enum.converters.diodetrr.trr_factor  diode_trr_factor=3  diode_trr=15 us  diode_Qrr=1500 s*uA
  MOSFETB2 : ee_lib/Semiconductors & Converters/Ideal Semiconductor Switch  port_option=ee.enum.controlport.ps  Ron=RdsOnPri_SI Ohm  Goff=GdsOffPri_SI 1/Ohm  Vth=VthPri_SI V  diode_param=ee.enum.semiconductors.protectionDiode.nodynamics  diode_Vf=VfPri_SI V  diode_Ron=RdPri_SI Ohm  diode_Goff=GdPri_SI 1/Ohm  diode_C=50e-9 F  diode_iRM=-235 A  diode_iF=300 A  diode_idot=-50 A/us  diode_trr_param=ee.enum.converters.diodetrr.trr_factor  diode_trr_factor=3  diode_trr=15 us  diode_Qrr=1500 s*uA
  MOSFETPriA1 : ee_lib/Semiconductors & Converters/Ideal Semiconductor Switch  port_option=ee.enum.controlport.ps  Ron=RdsOnPri_SI Ohm  Goff=GdsOffPri_SI 1/Ohm  Vth=VthPri_SI V  diode_param=ee.enum.semiconductors.protectionDiode.nodynamics  diode_Vf=VfPri_SI V  diode_Ron=RdPri_SI Ohm  diode_Goff=GdPri_SI 1/Ohm  diode_C=50e-9 F  diode_iRM=-235 A  diode_iF=300 A  diode_idot=-50 A/us  diode_trr_param=ee.enum.converters.diodetrr.trr_factor  diode_trr_factor=3  diode_trr=15 us  diode_Qrr=1500 s*uA
  MOSFETPriA2 : ee_lib/Semiconductors & Converters/Ideal Semiconductor Switch  port_option=ee.enum.controlport.ps  Ron=RdsOnPri_SI Ohm  Goff=GdsOffPri_SI 1/Ohm  Vth=VthPri_SI V  diode_param=ee.enum.semiconductors.protectionDiode.nodynamics  diode_Vf=VfPri_SI V  diode_Ron=RdPri_SI Ohm  diode_Goff=GdPri_SI 1/Ohm  diode_C=50e-9 F  diode_iRM=-235 A  diode_iF=300 A  diode_idot=-50 A/us  diode_trr_param=ee.enum.converters.diodetrr.trr_factor  diode_trr_factor=3  diode_trr=15 us  diode_Qrr=1500 s*uA
  MOSFETSecA1 : ee_lib/Semiconductors & Converters/Ideal Semiconductor Switch  port_option=ee.enum.controlport.ps  Ron=RdsOnSec_SI Ohm  Goff=GdsOffSec_SI 1/Ohm  Vth=VthSec_SI V  diode_param=ee.enum.semiconductors.protectionDiode.nodynamics  diode_Vf=VfSec_SI V  diode_Ron=RdSec_SI Ohm  diode_Goff=GdSec_SI 1/Ohm  diode_C=50e-9 F  diode_iRM=-235 A  diode_iF=300 A  diode_idot=-50 A/us  diode_trr_param=ee.enum.converters.diodetrr.trr_factor  diode_trr_factor=3  diode_trr=15 us  diode_Qrr=1500 s*uA
  MOSFETSecA2 : ee_lib/Semiconductors & Converters/Ideal Semiconductor Switch  port_option=ee.enum.controlport.ps  Ron=RdsOnSec_SI Ohm  Goff=GdsOffSec_SI 1/Ohm  Vth=VthSec_SI V  diode_param=ee.enum.semiconductors.protectionDiode.nodynamics  diode_Vf=VfSec_SI V  diode_Ron=RdSec_SI Ohm  diode_Goff=GdSec_SI 1/Ohm  diode_C=50e-9 F  diode_iRM=-235 A  diode_iF=300 A  diode_idot=-50 A/us  diode_trr_param=ee.enum.converters.diodetrr.trr_factor  diode_trr_factor=3  diode_trr=15 us  diode_Qrr=1500 s*uA
  MOSFETSecB1 : ee_lib/Semiconductors & Converters/Ideal Semiconductor Switch  port_option=ee.enum.controlport.ps  Ron=RdsOnSec_SI Ohm  Goff=GdsOffSec_SI 1/Ohm  Vth=VthSec_SI V  diode_param=ee.enum.semiconductors.protectionDiode.nodynamics  diode_Vf=VfSec_SI V  diode_Ron=RdSec_SI Ohm  diode_Goff=GdSec_SI 1/Ohm  diode_C=50e-9 F  diode_iRM=-235 A  diode_iF=300 A  diode_idot=-50 A/us  diode_trr_param=ee.enum.converters.diodetrr.trr_factor  diode_trr_factor=3  diode_trr=15 us  diode_Qrr=1500 s*uA
  MOSFETSecB2 : ee_lib/Semiconductors & Converters/Ideal Semiconductor Switch  port_option=ee.enum.controlport.ps  Ron=RdsOnSec_SI Ohm  Goff=GdsOffSec_SI 1/Ohm  Vth=VthSec_SI V  diode_param=ee.enum.semiconductors.protectionDiode.nodynamics  diode_Vf=VfSec_SI V  diode_Ron=RdSec_SI Ohm  diode_Goff=GdSec_SI 1/Ohm  diode_C=50e-9 F  diode_iRM=-235 A  diode_iF=300 A  diode_idot=-50 A/us  diode_trr_param=ee.enum.converters.diodetrr.trr_factor  diode_trr_factor=3  diode_trr=15 us  diode_Qrr=1500 s*uA
  Simulink-PS Converter{,1..7} (8 alike) : nesl_utility/Simulink-PS Converter  PhysicalDomain=network_engine_domain  SubClassName=ps_input  LeftPortType=input  RightPortType=output  PseudoPeriodic=off  Frequencies=[]  NoiseDistribution=none  NoiseParameters=[]  Unit=1  AffineConversion=off  FilteringAndDerivatives=provide  SimscapeFilterOrder=1  InputFilterTimeConstant=0.001  UdotUserProvided=0
  Transformer : ee_lib/Passive/Transformers/Mutual Inductor  L1=Lm_SI+Llk1_SI H  L2=Lm_SI/turnsRatio^2+Llk2_SI H  k=Lm_SI/sqrt((Lm_SI+Llk1_SI)*(Lm_SI+turnsRatio^2*Llk2_SI))  L_tol=0  enable_L1_tol=ee.enum.toleranceApplication.none  L1_tol_distribution=ee.enum.toleranceDistribution.uniform  L1_nSigma=4  enable_L2_tol=ee.enum.toleranceApplication.none  L2_tol_distribution=ee.enum.toleranceDistribution.uniform  L2_nSigma=4  r=[RLlk1_SI, RLlk2_SI] Ohm  g=[1e-09, 1e-09] 1/Ohm  enable_operating_limits=ee.enum.enable.no  operating_limit_action=ee.enum.passive.reportOpLim.warn  max_working_current=1 A  power_rating=1 W  iL1_specify=off  iL1_priority=High  iL1=0 A  iL1_nominal_specify=off  iL1_nominal_value=1  iL1_nominal_unit=A  iL2_specify=off  iL2_priority=High  iL2=0 A  iL2_nominal_specify=off  iL2_nominal_value=1  iL2_nominal_unit=A
  VinSens : Subsystem
      mask Display: disp('V')
  VoutSens : Subsystem
      settings: PortSchema="{\"entries\":[{\"content\":{\"sides\":[{\"content\":{\"connectorIds\":[\"LConn1\"]},\"type\":\"ConnectorPlacement.EquallySpacedRectSide\",\"uuid\":\"da66b42d-39ba-4e5d-9b19-dc680792542d\"},{\"content\":{\"connectorIds\":[\"RConn1\",\"Out1\"],\"side\":\"RIGHT\"},\"type\":\"ConnectorPlacement.EquallySpacedRectSide\",\"uuid\":\"9a34d54a-b1f0-405a-82c9-4333c7864e33\"},{\"content\":{\"side\":\"TOP\"},\"type\":\"ConnectorPlacement.EquallySpacedRectSide\",\"uuid\":\"3d98f795-d173-4072-aa84-47617691d0d7\"}]},\"type\":\"ConnectorPlacement.EquallySpacedConnector\",\"uuid\":\"cc1a3107-18f6-4c4b-a82f-56637250e4a4\"}],\"packageUris\":[\"http://schema.mathworks.com/mf0/Connector/R2020b\"],\"version\":\"1.0\"}"
      mask Display: disp('V')
  Vin+ : PMIOPort  Side=Left
  Vin- : PMIOPort  Port=2  Side=Left
  Vout+ : PMIOPort  Port=3  Side=Right
  Vout- : PMIOPort  Port=4  Side=Right
  Out Bus Element1 : Outport  PortName=meas  Element=Ip [A]
  Out Bus Element2 : Outport  PortName=meas  Element=Is [A]
  Out Bus Element3 : Outport  PortName=meas  Element=Vin [V]
  Out Bus Element4 : Outport  PortName=meas  Element=Vout [V]
  Out Bus Element5 : Outport  PortName=meas  Element=Iin [A]
  Out Bus Element6 : Outport  PortName=meas  Element=Iout [A]
  wires:
  Gs/1 -> Demux1/1
  [G8] -> Simulink-PS Converter7/1
  [G7] -> Simulink-PS Converter6/1
  [G6] -> Simulink-PS Converter5/1
  [G5] -> Simulink-PS Converter4/1
  [G4] -> Simulink-PS Converter3/1
  [G3] -> Simulink-PS Converter2/1
  [G1] -> Simulink-PS Converter/1
  VoutSens/1(V) -> Out Bus Element4/1
  VinSens/1(V) -> Out Bus Element3/1
  Is/1(I) -> Out Bus Element2/1
  Ip/1(I) -> Out Bus Element1/1
  Iout/1(I) -> Out Bus Element6/1
  Iin/1(I) -> Out Bus Element5/1
  [G2] -> Simulink-PS Converter1/1
  Demux1/4 -> [G8]
  Demux1/3 -> [G7]
  Demux1/2 -> [G6]
  Demux1/1 -> [G5]
  Demux/4 -> [G4]
  Demux/3 -> [G3]
  Demux/2 -> [G2]
  Demux/1 -> [G1]
  Gp/1 -> Demux/1
  connections:
  Iin/RConn1 -- MOSFETB1/RConn1 -- MOSFETPriA1/RConn1
  VoutSens/LConn1 -- Vout+/RConn1 -- Iout/RConn1
  MOSFETSecA2/RConn2 -- Co/RConn1 -- Vout-/RConn1 -- VoutSens/RConn1 -- MOSFETSecB2/RConn2
  Simulink-PS Converter7/RConn1 -- MOSFETSecB2/LConn1
  Simulink-PS Converter6/RConn1 -- MOSFETSecB1/LConn1
  MOSFETSecB2/RConn1 -- Transformer/RConn2 -- MOSFETSecB1/RConn2
  MOSFETSecB1/RConn1 -- Co/LConn1 -- Iout/LConn1 -- MOSFETSecA1/RConn1
  Simulink-PS Converter5/RConn1 -- MOSFETSecA2/LConn1
  Simulink-PS Converter4/RConn1 -- MOSFETSecA1/LConn1
  Is/LConn1 -- Transformer/RConn1
  Transformer/LConn1 -- Lr/RConn1
  Ip/RConn1 -- Lr/LConn1
  MOSFETSecA2/RConn1 -- Is/RConn1 -- MOSFETSecA1/RConn2
  MOSFETPriA2/RConn2 -- MOSFETB2/RConn2 -- Vin-/RConn1 -- VinSens/RConn1
  VinSens/LConn1 -- Iin/LConn1 -- Vin+/RConn1
  MOSFETB2/RConn1 -- Transformer/LConn2 -- MOSFETB1/RConn2
  Simulink-PS Converter3/RConn1 -- MOSFETB2/LConn1
  Simulink-PS Converter2/RConn1 -- MOSFETB1/LConn1
  Simulink-PS Converter1/RConn1 -- MOSFETPriA2/LConn1
  Simulink-PS Converter/RConn1 -- MOSFETPriA1/LConn1
  MOSFETPriA2/RConn1 -- Ip/LConn1 -- MOSFETPriA1/RConn2

== system ConverterLibrary/Power Converter Plant/Soft-Switching Converters/LLC Converter/LLC Primary Inverter and Resonant Tank/LLC Detailed Model ==
  G : Inport
  Inverter : Subsystem
      settings: PortSchema="{\"entries\":[{\"content\":{\"sides\":[{\"content\":{\"connectorIds\":[\"LConn1\",\"LConn2\"]},\"type\":\"ConnectorPlacement.EquallySpacedRectSide\",\"uuid\":\"5f98eff0-54e4-47a8-aeeb-0279cba14f26\"},{\"content\":{\"connectorIds\":[\"RConn1\",\"RConn2\"],\"side\":\"RIGHT\"},\"type\":\"ConnectorPlacement.EquallySpacedRectSide\",\"uuid\":\"71acbbb6-1fc8-426c-b389-5d494eb18bfd\"},{\"content\":{\"connectorIds\":[\"In1\",\"Out1\"],\"side\":\"TOP\"},\"type\":\"ConnectorPlacement.EquallySpacedRectSide\",\"uuid\":\"dc77ee05-1f57-4323-bfda-b0076e2d1ee5\"}]},\"type\":\"ConnectorPlacement.EquallySpacedConnector\",\"uuid\":\"8d0b8c05-d5c5-4033-af60-ebdb639bdc40\"}],\"packageUris\":[\"http://schema.mathworks.com/mf0/Connector/R2020b\"],\"version\":\"1.0\"}"
  Resonant Tank : Subsystem
      settings: PortSchema="{\"entries\":[{\"content\":{\"sides\":[{\"content\":{\"connectorIds\":[\"LConn1\",\"LConn2\"]},\"type\":\"ConnectorPlacement.EquallySpacedRectSide\",\"uuid\":\"d505f362-3b8e-4dee-9b5b-731d75550efb\"},{\"content\":{\"connectorIds\":[\"RConn1\",\"RConn2\",\"RConn3\"],\"side\":\"RIGHT\"},\"type\":\"ConnectorPlacement.EquallySpacedRectSide\",\"uuid\":\"66ab4b84-9b7a-404b-b3f6-3ac1c371ea42\"},{\"content\":{\"connectorIds\":[\"Out1\"],\"side\":\"TOP\"},\"type\":\"ConnectorPlacement.EquallySpacedRectSide\",\"uuid\":\"00605859-d490-4a3b-aace-391362dfba7e\"}]},\"type\":\"ConnectorPlacement.EquallySpacedConnector\",\"uuid\":\"a210fe68-7181-499f-8e1c-ccfe71b42a4c\"}],\"packageUris\":[\"http://schema.mathworks.com/mf0/Connector/R2020b\"],\"version\":\"1.0\"}"
      mask Display: image('LLCTransformerIcon.png');
  + : PMIOPort  Side=Left
  P2+ : PMIOPort  Port=2  Side=Right
  N2 : PMIOPort  Port=3  Side=Right
  - : PMIOPort  Port=4  Side=Left
  P2- : PMIOPort  Port=5  Side=Right
  measInv : Outport
  measTank : Outport  Port=2
  wires:
  Resonant Tank/1(meas) -> measTank/1  "ResonantTank"
  Inverter/1(meas) -> measInv/1  "Inverter"
  G/1 -> Inverter/1(G)
  connections:
  Resonant Tank/RConn2 -- N2/RConn1
  +/RConn1 -- Inverter/LConn1
  Resonant Tank/RConn1 -- P2+/RConn1
  Resonant Tank/LConn2 -- Inverter/RConn2
  Resonant Tank/RConn3 -- P2-/RConn1
  Resonant Tank/LConn1 -- Inverter/RConn1
  -/RConn1 -- Inverter/LConn2
